simulink subsystem "acc"  (R2025b)
settings: Solver=VariableStepAuto  StartTime=0.0  StopTime=10.0  RelTol=1e-3
settings Model: Creator=sanborkl  LastModifiedBy=sanborkl

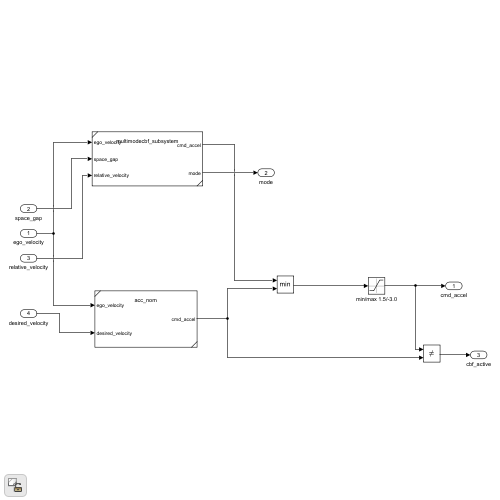
[thumbnail: Simulink's stored preview of the top-level diagram]
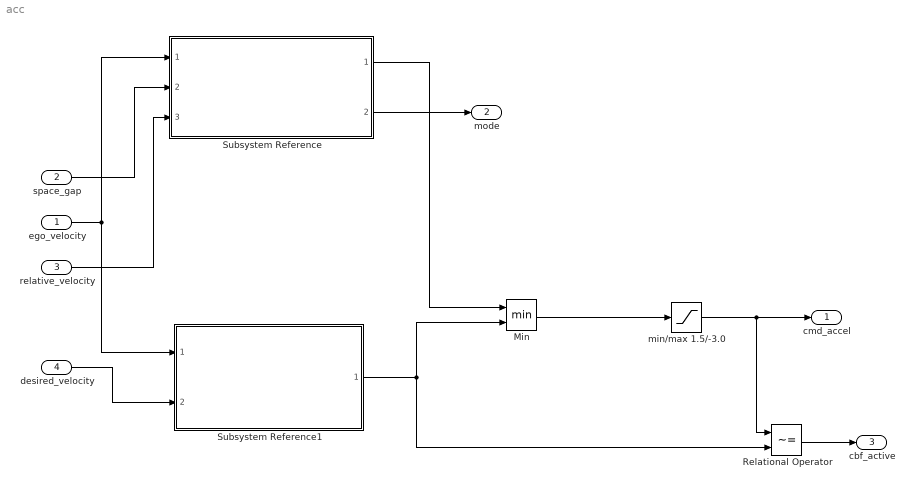
== system acc ==
  ego_velocity : Inport
  space_gap : Inport  Port=2
  relative_velocity : Inport  Port=3
  desired_velocity : Inport  Port=4
  Min : MinMax  Inputs=2
  Relational Operator : RelationalOperator  Operator=~=  OutDataTypeStr=boolean  RndMeth=Simplest  InputSameDT=off
  Subsystem Reference : Subsystem  ReferencedSubsystem=multimodecbf_subsystem
  Subsystem Reference1 : Subsystem  ReferencedSubsystem=acc_nom
  min/max 1.5/-3.0 : Saturate  UpperLimit=1.5  LowerLimit=-3.0
  cmd_accel : Outport
  mode : Outport  Port=2
  cbf_active : Outport  Port=3
  wires:
  Subsystem Reference1/1 -> Min/2, Relational Operator/2
  Relational Operator/1 -> cbf_active/1
  Subsystem Reference/2 -> mode/1
  desired_velocity/1 -> Subsystem Reference1/2
  ego_velocity/1 -> Subsystem Reference1/1, Subsystem Reference/1
  space_gap/1 -> Subsystem Reference/2
  relative_velocity/1 -> Subsystem Reference/3
  Subsystem Reference/1 -> Min/1
  Min/1 -> min/max 1.5/-3.0/1
  min/max 1.5/-3.0/1 -> cmd_accel/1, Relational Operator/1
